simulink model "TankModel"  (R2024a)
settings: Solver=VariableStepAuto  StartTime=0.0  StopTime=2000  RelTol=1e-3
values from neighbouring files (symbols this model uses):
  A1 = 0.02    [matlab.mat]    (also in params.m)
  A2 = 0.02    [matlab.mat]    (also in params.m)
  h1_ss = h2_ss    (= 0.2)    [params.m]
  h2_ss = 0.2    [params.m]
  k1 = 0.000132883407542    [matlab.mat]    (also in params.m = Cd1*a1*sqrt(2*g))
  k2 = 0.000132883407542    [matlab.mat]    (also in params.m = Cd2*a2*sqrt(2*g))
  Kd = K - Kp/N    (= 0.021748502208)    [params.m]
  kd_extra = 0.25*k2    [params.m]
  Ki = K*z^2    (= 1.65525552e-06)    [params.m]
  Kp = 0.000186    [design_controller.m]    (also in params.m = 0.0004125748896)
  Nf = N    (= 0.05)    [params.m]
  Qin_ss = Q1_ss    [params.m]
  Qmax = 9e-5    (= 9e-05)    [params.m]
  u_max = Qmax - Qin_ss    [params.m]
  u_min = -Qin_ss    [params.m]
libraries: slpidlib x1
settings Model: Creator=User  LastModifiedBy=User

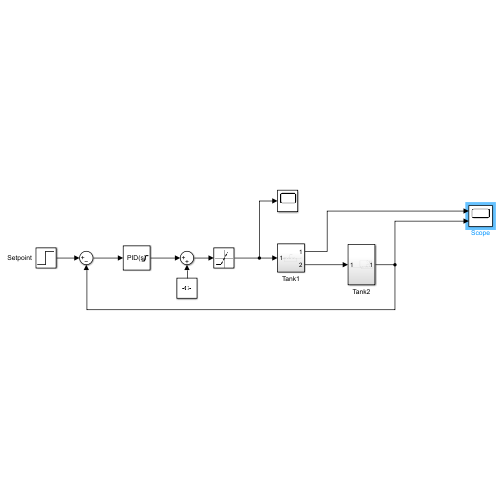
[thumbnail: Simulink's stored preview of the top-level diagram]
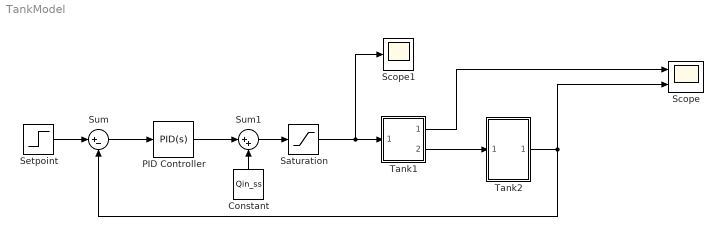
== system TankModel ==
  Constant : Constant  Value=Qin_ss
  PID Controller : slpidlib/PID Controller  Controller=PID  Form=Parallel  TimeDomain=Continuous-time  UseExternalTs=off  SampleTime=-1  IntegratorMethod=Forward Euler  FilterMethod=Forward Euler  ControllerParametersSource=internal  P=Kp  I=Ki  UseKiTs=off  D=Kd  UseExternalDerivativeSource=off  N=Nf  UseFilter=on  TunerSelectOption=Transfer Function Based (PID Tuner App)  InitialConditionSource=internal  InitialConditionForIntegrator=0  InitialConditionForFilter=0  DifferentiatorICPrevScaledInput=0  ExternalReset=none  TrackingMode=off  Kt=1  LimitOutput=on  SatLimitsSource=internal  UpperSaturationLimit=u_max  LowerSaturationLimit=u_min  LinearizeAsGain=on  AntiWindupMode=clamping  Kb=1  LimitIntegrator=off  UpperIntegratorSaturationLimit=inf  LowerIntegratorSaturationLimit=-inf  POutMin=[]  POutMax=[]  IOutMin=[]  IOutMax=[]  DOutMin=[]  DOutMax=[]  NOutMin=[]  NOutMax=[]  SumOutMin=[]  SumOutMax=[]  SaturationOutMin=[]  SaturationOutMax=[]  PParamMin=[]  PParamMax=[]  IParamMin=[]  IParamMax=[]  DParamMin=[]  DParamMax=[]  NParamMin=[]  NParamMax=[]  KbParamMin=[]  KbParamMax=[]  KtParamMin=[]  KtParamMax=[]  KbOutMin=[]  KbOutMax=[]  KtOutMin=[]  KtOutMax=[]  IntegratorOutMin=[]  IntegratorOutMax=[]  FilterOutMin=[]  FilterOutMax=[]  SumI1OutMin=[]  SumI1OutMax=[]  SumI2OutMin=[]  SumI2OutMax=[]  SumI3OutMin=[]  SumI3OutMax=[]  SumI4OutMin=[]  SumI4OutMax=[]  SumDOutMin=[]  SumDOutMax=[]  DifferentiatorOutMin=[]  DifferentiatorOutMax=[]  FilterDiffOutCoefMin=[]  FilterDiffOutCoefMax=[]  ReciprocalOutMin=[]  ReciprocalOutMax=[]  SumDenOutMin=[]  SumDenOutMax=[]  SumNumOutMin=[]  SumNumOutMax=[]  DivideOutMin=[]  DivideOutMax=[]  UdiffTsProdOutMin=[]  UdiffTsProdOutMax=[]  NTsProdOutMin=[]  NTsProdOutMax=[]  UintegralTsProdOutMin=[]  UintegralTsProdOutMax=[]  UngainTsProdOutMin=[]  UngainTsProdOutMax=[]  ClampingZeroOutDataTypeStr=Inherit: Inherit via back propagation  ClampingZeroOutMin=[]  ClampingZeroOutMax=[]  FilterDenConstantOutDataTypeStr=Inherit: Inherit via back propagation  FilterDenConstantOutMin=[]  FilterDenConstantOutMax=[]  PCopyOutDataTypeStr=Inherit: Inherit via back propagation  PCopyOutMin=[]  PCopyOutMax=[]  NCopyOutDataTypeStr=Inherit: Inherit via back propagation  NCopyOutMin=[]  NCopyOutMax=[]  IntegratorContinuousStateAttributes=''  IntegratorStateMustResolveToSignalObject=off  IntegratorRTWStateStorageClass=Auto  FilterContinuousStateAttributes=''  FilterStateMustResolveToSignalObject=off  FilterRTWStateStorageClass=Auto  ParallelPVariant=InternalParameters  IdealPVariant=Disabled  IVariant=InternalParameters  DVariant=InternalParameters  IntegratorVariant=Continuous  SatVariant=Enabled  AWVariant=ContClampingParallel  PCopyVariant=Disabled  TRVariant=Disabled  FdbkBlocksVariant=Forward  IdealPFdbkVariant=Disabled  SatFdbkVariant=Disabled  DerivativeFilterVariant=ContFilter  NVariant=InternalParameters  NCopyVariant=Disabled  FilterICVariant=InternalICsFilter  IntegratorICVariant=InternalICs  ExternalResetVariant=Disabled  TRSumVariant=Passthrough  SumFdbkVariant=Disabled  SumVariant=Sum_PID  TsampFilterVariant=InternalTs  TsampNgainVariant=Passthrough  TsampIntegralVariant=Disabled_SignalSpec  ExternalSaturationOutDataTypeStr=Inherit: Same as second input  DerivativeSourceVariant=ErrorSignal
  Saturation : Saturate  UpperLimit=Qmax  LowerLimit=0
  Scope : Scope  NumInputPorts=2
  Scope1 : Scope
  Setpoint : Step  Time=100  Before=0.2  After=0.2  SampleTime=0
  Sum : Sum  Inputs=|+-
  Sum1 : Sum  Inputs=|++
  Tank1 : Subsystem
  Tank2 : Subsystem
  wires:
  Tank2/1(Out1) -> Sum/2, Scope/2
  Tank1/2(Out2) -> Tank2/1(In1)
  Tank1/1(Out1) -> Scope/1
  Setpoint/1 -> Sum/1
  Constant/1 -> Sum1/2
  Sum1/1 -> Saturation/1
  Saturation/1 -> Scope1/1, Tank1/1(In1)
  Sum/1 -> PID Controller/1
  PID Controller/1 -> Sum1/1

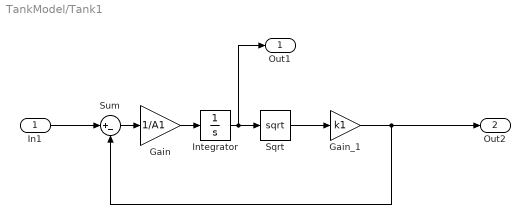
== system TankModel/Tank1 ==
  In1 : Inport
  Gain : Gain  Gain=1/A1
  Gain_1 : Gain  Gain=k1
  Integrator : Integrator  InitialCondition=h1_ss
  Sqrt : Sqrt
  Sum : Sum  Inputs=|+-
  Out1 : Outport
  Out2 : Outport  Port=2
  wires:
  In1/1 -> Sum/1
  Gain_1/1 -> Out2/1, Sum/2
  Integrator/1 -> Out1/1, Sqrt/1
  Sqrt/1 -> Gain_1/1
  Sum/1 -> Gain/1
  Gain/1 -> Integrator/1

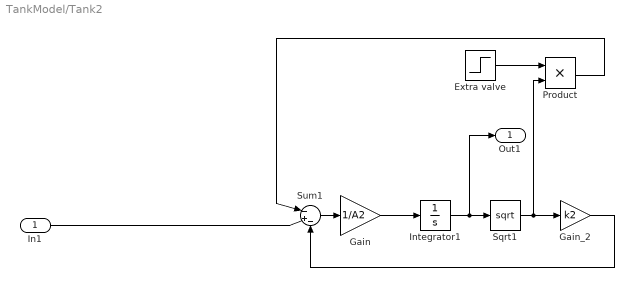
== system TankModel/Tank2 ==
  In1 : Inport
  Extra valve : Step  Time=600  After=kd_extra  SampleTime=0
  Gain : Gain  Gain=1/A2
  Gain_2 : Gain  Gain=k2
  Integrator1 : Integrator  InitialCondition=h2_ss
  Product : Product
  Sqrt1 : Sqrt
  Sum1 : Sum  Inputs=|-+-
  Out1 : Outport
  wires:
  Integrator1/1 -> Out1/1, Sqrt1/1
  Sqrt1/1 -> Product/2, Gain_2/1
  Sum1/1 -> Gain/1
  Gain/1 -> Integrator1/1
  In1/1 -> Sum1/2
  Gain_2/1 -> Sum1/3
  Extra valve/1 -> Product/1
  Product/1 -> Sum1/1
